simulink model "afe_inv_ttype_psm"  (R2026a)
settings: Solver=ode23tb  StopTime=simlength  FixedStep=tc  MaxStep=glb_time.tc
values from neighbouring files (symbols this model uses):
  afe_ctrl = ctrl_afe_setup(glb_time.ts_afe, grid_emu.omega_grid_nom)    [init_model.m]
  afe_pwm_phase_shift_mod1 = 0    [init_model.m]
  DThs_init = 0    [init_model.m]
  filters = setup_global_filters(glb_time.ts_afe, glb_time.ts_inv, glb_time.ts_dab, glb_time.tc)    [init_model.m]
  frt_data = frt_settings(test_index, test_subindex, asymmetric_error_type,      enable_frt_1, enable_frt_2, start_time_LVRT, deepPOSxi, deepPOSeta, deepNEGxi, deepNEGeta)    [init_model.m]
  glb_time = timing_setup(fpwm_afe, trgo_afe, fpwm_inv, trgo_inv, fpwm_single_phase_inv, trgo_single_phase_inv, fpwm_dab, trgo_dab,      fpwm_psfbc, trgo_psfbc, fpwm_isop_rail, trgo_isop_rail, fpwm_cllc, trgo_cllc, t_measure, tc_factor, tc_decimation, delay_pwm, dead_time_afe,      dead_time_inv, dead_time_single_phase_inv, dead_time_dab, dead_time_psfbc, dead_time_isop_rail, dead_time_cllc)    [init_model.m]
  grid_emu = grid_three_phase_emulator('Dyn11', delta_star, grid_nominal_power, application_voltage, us1, us2, fgrid,                  eq_grid_inductance, eq_grid_resistance, eta, ucc, i1m, p_iron, n1, n2, core_area, core_length, mur,                  up_xi_pu_ref, up_eta_pu_ref, un_xi_pu_ref, un_eta_pu_ref)    [init_model.m]
  i_react_pos_ref_2 = -ixi_ref_mod1*tan(acos(0.95))    [init_model.m]
  i_react_pos_ref_3 = ixi_ref_mod1*tan(acos(0.95))    [init_model.m]
  ixi_ref_mod1 = -0.85    [init_model.m]
  ki_align = 18    [init_model.m]
  kp_align = 0.25    [init_model.m]
  lim_down_align = -0.05    [init_model.m]
  lim_up_align = 0.05    [init_model.m]
  mavarage_filter_frequency_base_order = 2    [init_model.m]
  omega_m_sim = psm.omega_m_bez    [init_model.m]
  psm = psm_calculus()    [init_model.m]
  psm_ctrl = ctrl_pmsm_setup(glb_time.ts_inv, psm.omega_bez, u_psm_scale, psm.Jm_norm)    [init_model.m]
  simlength = 1.75    [init_model.m]
  Tambient = 40    [init_model.m]
  time_aux_power_supply_fault = 1e3    (= 1000)    [init_model.m]
  time_gain_afe_module_1 = 1.0002    [init_model.m]
  time_gain_inv_module_2 = 1.001    [init_model.m]
  time_i_react_pos_ref_1 = start_time_LVRT + error_length + 0.335    [init_model.m]
  time_i_react_pos_ref_2 = time_i_react_pos_ref_1 + 0.5    (= 0.5)    [init_model.m]
  time_start_motor_control = 0.25    [init_model.m]
  torque_overload_factor = 1    [init_model.m]
  u_cm_comp_mod1 = 0    [init_model.m]
  u_psm_scale_ekf = sqrt(3)/2 * 2/3 * hwdata.inv.udc_nom/psm.ubez    [init_model.m]
undefined symbols (not defined in the file or in its folder): hwdata, magnitude, omega_m_bez, rpm_base, torque_base
libraries: fl_lib x74, nesl_utility x43, moving_average_filter x10, moving_average_filter_cc x8, discrete_time_low_pass_filter x4, sl_discontinuities x3, single_phase_transformer_lib x3, linear_double_integrator_observer_ccaller x2, threephase_inductor_lib x2, dclink_for_three_levels x2, three_phase_three_level_ttype_inverter_ideal_switch_based_model x2, cstblocks_lti x2
(part 1 of 9)
settings Model: SimulationMode=accelerator  Creator=dbagn  LastModifiedBy=dbagn
settings SolverCC: NumberNewtonIterations=3.0  ZeroCrossControl=DisableAll  SolverResetMethod=Robust
settings SFSimCC: CustomCodeUndefinedFunction=ThrowError  DefaultCustomCodeDeterministicFunctions=All
settings SFSimCC: SimCustomHeaderCode=|
  | #include "rpi.h"
  | #include "mavgflt.h"
  | #include "mavgflt_simulink.h"
  | #include "mavgflts.h"
  | #include "mavgflts_simulink.h"
  | #include "dsmavgflt.h"
  | #include "dsmavgflt_simulink.h"
  | #include "bemf_obsv.h"
  | #include "bemf_obsv_simulink.h"
  | #include "bemf_obsv_load_est.h"
  | #include "bemf_obsv_load_est_simulink.h"
  | #include "dqvector_pi.h"
  | #include "dqvector_pi_simulink.h"
  | #include "sv_pwm_simulink.h"
  | #include "sv_pwm.h"
  | #include "sv_pwm_cm_simulink.h"
  | #include "sv_pwm_cm.h"
  | #include "first_harmonic_tracker.h"
  | #include "first_harmonic_tracker_simulink.h"
  | #include "dqpll_thyr.h"
  | #include "dqpll_thyr_simulink.h"
  | #include "dqpll_grid.h"
  | #include "dqpll_grid_simulink.h"
  | #include "linear_double_integrator_observer_simulink.h"
  | #include "linear_double_integrator_observer.h"
settings SFSimCC: SimUserSources=|
  | "rpi.c"
  | "mavgflt_simulink.c"
  | "mavgflt.c"
  | "mavgflts_simulink.c"
  | "mavgflts.c"
  | "dsmavgflt_simulink.c"
  | "dsmavgflt.c"
  | "bemf_obsv_simulink.c"
  | "bemf_obsv.c"
  | "bemf_obsv_load_est_simulink.c"
  | "bemf_obsv_load_est.c"
  | "dqvector_pi.c"
  | "dqvector_pi_simulink.c"
  | "sv_pwm_simulink.c"
  | "sv_pwm.c"
  | "sv_pwm_cm_simulink.c"
  | "sv_pwm_cm.c"
  | "first_harmonic_tracker_simulink.c"
  | "first_harmonic_tracker.c"
  | "dqpll_thyr_simulink.c"
  | "dqpll_thyr.c"
  | "dqpll_grid_simulink.c"
  | "dqpll_grid.c"
  | "linear_double_integrator_observer_simulink.c"
  | "linear_double_integrator_observer.c"
settings SFSimCC: SimUserIncludeDirs=|
  | include
  | src
settings SimscapeCC: SimscapeNominalValues="[{\"value\":\"1\",\"unit\":\"A\"},{\"value\":\"1\",\"unit\":\"bar\"},{\"value\":\"1\",\"unit\":\"cm^2\"},{\"value\":\"1\",\"unit\":\"cm^3/s\"},{\"value\":\"1\",\"unit\":\"kJ/kg\"},{\"value\":\"1\",\"unit\":\"kW\"},{\"value\":\"1\",\"unit\":\"l\"},{\"value\":\"1\",\"unit\":\"N\"},{\"value\":\"1\",\"unit\":\"N*m\"},{\"value\":\"1\",\"unit\":\"V\"}]"  SimscapeLogType=none  SimscapeLogDataHistory=5000.0

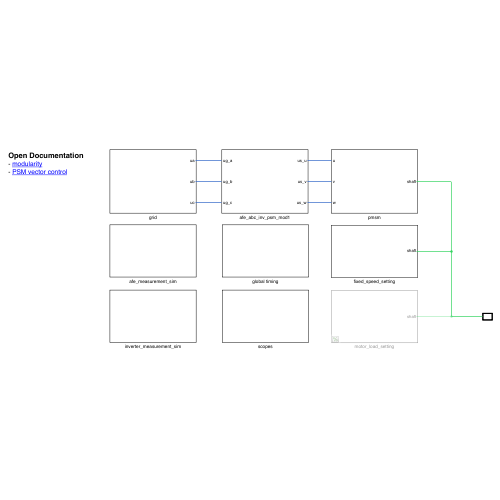
[thumbnail: Simulink's stored preview of the top-level diagram]
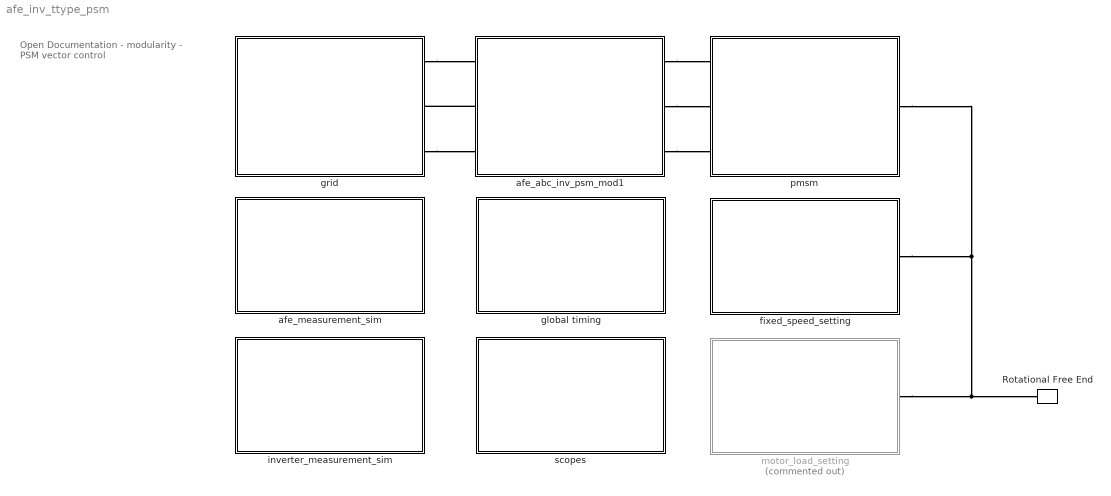
== system afe_inv_ttype_psm ==
  note: Open Documentation
      | - modularity
      | - PSM vector control
  Rotational Free End : fl_lib/Mechanical/Rotational Elements/Rotational Free End  w_specify=off  w_priority=None  w=0 rad/s  w_nominal_specify=off  w_nominal_value=1  w_nominal_unit=rad/s
  afe_abc_inv_psm_mod1 : Subsystem
  afe_measurement_sim : Subsystem
  fixed_speed_setting : Subsystem
  global timing : Subsystem
  grid : Subsystem
  inverter_measurement_sim : Subsystem
  motor_load_setting : Subsystem  Commented=on
  pmsm : Subsystem
  scopes : Subsystem
  connections:
  pmsm/RConn1 -- motor_load_setting/LConn1 -- Rotational Free End/LConn1 -- fixed_speed_setting/LConn1
  grid/RConn1 -- afe_abc_inv_psm_mod1/LConn1
  grid/RConn3 -- afe_abc_inv_psm_mod1/LConn3
  afe_abc_inv_psm_mod1/LConn2 -- grid/RConn2
  afe_abc_inv_psm_mod1/RConn2 -- pmsm/LConn2
  afe_abc_inv_psm_mod1/RConn1 -- pmsm/LConn1
  afe_abc_inv_psm_mod1/RConn3 -- pmsm/LConn3

== system afe_inv_ttype_psm/afe_abc_inv_psm_mod1 ==
  AFE_control : Subsystem
  LCL_filter : Subsystem
  afe : Subsystem
  brake : Subsystem
  inv_psm_mod1 : Subsystem
  ug_a : PMIOPort  Side=Left
  us_u : PMIOPort  Port=2  Side=Right
  ug_b : PMIOPort  Port=3  Side=Left
  us_v : PMIOPort  Port=4  Side=Right
  ug_c : PMIOPort  Port=5  Side=Left
  us_w : PMIOPort  Port=6  Side=Right
  wires:
  AFE_control/1(dabc_out) -> afe/1(dabc)
  connections:
  LCL_filter/LConn1 -- afe/LConn1
  LCL_filter/LConn2 -- afe/LConn2
  LCL_filter/LConn3 -- afe/LConn3
  LCL_filter/RConn1 -- ug_a/RConn1
  LCL_filter/RConn2 -- ug_b/RConn1
  LCL_filter/RConn3 -- ug_c/RConn1
  us_u/RConn1 -- inv_psm_mod1/RConn1
  us_v/RConn1 -- inv_psm_mod1/RConn2
  us_w/RConn1 -- inv_psm_mod1/RConn3
  inv_psm_mod1/LConn2 -- afe/RConn2
  afe/RConn1 -- brake/LConn1 -- inv_psm_mod1/LConn1
  afe/RConn3 -- brake/LConn2 -- inv_psm_mod1/LConn3

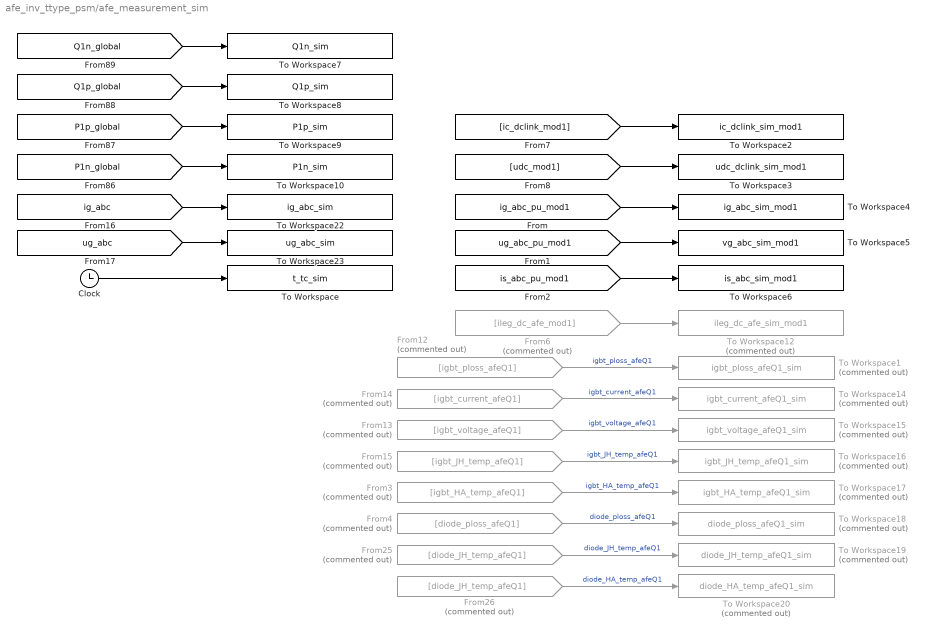
== system afe_inv_ttype_psm/afe_measurement_sim ==
  Clock : Clock
  From12 : From  Commented=on  GotoTag=igbt_ploss_afeQ1
  From13 : From  Commented=on  GotoTag=igbt_voltage_afeQ1
  From14 : From  Commented=on  GotoTag=igbt_current_afeQ1
  From15 : From  Commented=on  GotoTag=igbt_JH_temp_afeQ1
  From25 : From  Commented=on  GotoTag=diode_JH_temp_afeQ1
  From26 : From  Commented=on  GotoTag=diode_JH_temp_afeQ1
  From3 : From  Commented=on  GotoTag=igbt_HA_temp_afeQ1
  From4 : From  Commented=on  GotoTag=diode_ploss_afeQ1
  From6 : From  Commented=on  GotoTag=ileg_dc_afe_mod1
  To Workspace : ToWorkspace  VariableName=t_tc_sim  SampleTime=glb_time.tc
      settings: MaxDataPoints=glb_time.Nc
  To Workspace1 : ToWorkspace  Commented=on  VariableName=igbt_ploss_afeQ1_sim  SampleTime=glb_time.tc
      settings: MaxDataPoints=glb_time.Nc
  To Workspace10 : ToWorkspace  VariableName=P1n_sim  SampleTime=glb_time.ts_afe
      settings: MaxDataPoints=glb_time.Ns_afe
  To Workspace12 : ToWorkspace  Commented=on  VariableName=ileg_dc_afe_sim_mod1  SampleTime=glb_time.tc
      settings: MaxDataPoints=glb_time.Nc
  To Workspace14 : ToWorkspace  Commented=on  VariableName=igbt_current_afeQ1_sim  SampleTime=glb_time.tc
      settings: MaxDataPoints=glb_time.Nc
  To Workspace15 : ToWorkspace  Commented=on  VariableName=igbt_voltage_afeQ1_sim  SampleTime=glb_time.tc
      settings: MaxDataPoints=glb_time.Nc
  To Workspace16 : ToWorkspace  Commented=on  VariableName=igbt_JH_temp_afeQ1_sim  SampleTime=glb_time.tc
      settings: MaxDataPoints=glb_time.Nc
  To Workspace17 : ToWorkspace  Commented=on  VariableName=igbt_HA_temp_afeQ1_sim  SampleTime=glb_time.tc
      settings: MaxDataPoints=glb_time.Nc
  To Workspace18 : ToWorkspace  Commented=on  VariableName=diode_ploss_afeQ1_sim  SampleTime=glb_time.tc
      settings: MaxDataPoints=glb_time.Nc
  To Workspace19 : ToWorkspace  Commented=on  VariableName=diode_JH_temp_afeQ1_sim  SampleTime=glb_time.tc
      settings: MaxDataPoints=glb_time.Nc
  To Workspace2 : ToWorkspace  VariableName=ic_dclink_sim_mod1  SampleTime=glb_time.tc
      settings: MaxDataPoints=glb_time.Nc
  To Workspace20 : ToWorkspace  Commented=on  VariableName=diode_HA_temp_afeQ1_sim  SampleTime=glb_time.tc
      settings: MaxDataPoints=glb_time.Nc
  To Workspace22 : ToWorkspace  VariableName=ig_abc_sim  SampleTime=glb_time.tc
      settings: MaxDataPoints=glb_time.Nc
  To Workspace23 : ToWorkspace  VariableName=ug_abc_sim  SampleTime=glb_time.tc
      settings: MaxDataPoints=glb_time.Nc
  To Workspace3 : ToWorkspace  VariableName=udc_dclink_sim_mod1  SampleTime=glb_time.tc
      settings: MaxDataPoints=glb_time.Nc
  To Workspace4 : ToWorkspace  VariableName=ig_abc_sim_mod1  SampleTime=glb_time.tc
      settings: MaxDataPoints=glb_time.Nc
  To Workspace5 : ToWorkspace  VariableName=vg_abc_sim_mod1  SampleTime=glb_time.tc
      settings: MaxDataPoints=glb_time.Nc
  To Workspace6 : ToWorkspace  VariableName=is_abc_sim_mod1  SampleTime=glb_time.tc
      settings: MaxDataPoints=glb_time.Nc
  To Workspace7 : ToWorkspace  VariableName=Q1n_sim  SampleTime=glb_time.ts_afe
      settings: MaxDataPoints=glb_time.Ns_afe
  To Workspace8 : ToWorkspace  VariableName=Q1p_sim  SampleTime=glb_time.ts_afe
      settings: MaxDataPoints=glb_time.Ns_afe
  To Workspace9 : ToWorkspace  VariableName=P1p_sim  SampleTime=glb_time.ts_afe
      settings: MaxDataPoints=glb_time.Ns_afe
  wires:
  Clock/1 -> To Workspace/1
  [Q1n_global] -> To Workspace7/1
  [Q1p_global] -> To Workspace8/1
  [P1p_global] -> To Workspace9/1
  [P1n_global] -> To Workspace10/1
  [ug_abc] -> To Workspace23/1
  [ig_abc] -> To Workspace22/1
  [ug_abc_pu_mod1] -> To Workspace5/1
  [ig_abc_pu_mod1] -> To Workspace4/1
  From6/1 -> To Workspace12/1
  [udc_mod1] -> To Workspace3/1
  [ic_dclink_mod1] -> To Workspace2/1
  [is_abc_pu_mod1] -> To Workspace6/1
  From13/1 -> To Workspace15/1  "igbt_voltage_afeQ1"
  From3/1 -> To Workspace17/1  "igbt_HA_temp_afeQ1"
  From4/1 -> To Workspace18/1  "diode_ploss_afeQ1"
  From25/1 -> To Workspace19/1  "diode_JH_temp_afeQ1"
  From12/1 -> To Workspace1/1  "igbt_ploss_afeQ1"
  From26/1 -> To Workspace20/1  "diode_HA_temp_afeQ1"
  From14/1 -> To Workspace14/1  "igbt_current_afeQ1"
  From15/1 -> To Workspace16/1  "igbt_JH_temp_afeQ1"

== system afe_inv_ttype_psm/fixed_speed_setting ==
  Ideal Angular Velocity Source : fl_lib/Mechanical/Mechanical Sources/Ideal Angular Velocity Source
  Mechanical Rotational Reference : fl_lib/Mechanical/Rotational Elements/Mechanical Rotational Reference
  PS Step1 : fl_lib/Physical Signals/Sources/PS Step  step_time=0.025 s  initial_value=0 rpm  final_value=rpm_sim rpm
  PS Transfer Function : fl_lib/Physical Signals/Linear Operators/PS Transfer Function  transfer_function_type=foundation.enum.transfer_function_type.lag  T=0.1 s  T1=2 s  T2=1 s  reset_method=foundation.enum.IntegratorResetSpec.None  initial_condition_spec=foundation.enum.IntegratorICSpec.Internal  y0=0 rpm
  shaft : PMIOPort  Side=Left
  connections:
  Mechanical Rotational Reference/LConn1 -- Ideal Angular Velocity Source/RConn2
  PS Step1/RConn1 -- PS Transfer Function/LConn1
  PS Transfer Function/RConn1 -- Ideal Angular Velocity Source/RConn1
  Ideal Angular Velocity Source/LConn1 -- shaft/RConn1

== system afe_inv_ttype_psm/global timing ==
  Unit Delay : UnitDelay  SampleTime=glb_time.tc
  Unit Delay1 : UnitDelay  SampleTime=glb_time.tc
  time_afe1 : Subsystem  mask{k=time_gain_afe_module_1}
      mask prompts: k "Time Gain"
      mask Display:
      | disp('time-gen');
      | port_label('input', 1, 'crt');
      | port_label('output', 1, 'tout');
  time_afe3 : Subsystem  mask{k=1}
      mask prompts: k "Time Gain"
      mask Display:
      | disp('time-gen');
      | port_label('output', 1, 'tout');
  time_inv1 : Subsystem  mask{k=time_gain_inv_module_2}
      mask prompts: k "Time Gain"
      mask Display:
      | disp('time-gen');
      | port_label('input', 1, 'crt');
      | port_label('output', 1, 'tout');
  tag scope: time_afe_module_1=global, time_inv_module_1=global, time_master=global
  wires:
  time_afe1/1(Out1) -> [time_afe_module_1]
  time_inv1/1(Out1) -> [time_inv_module_1]
  time_afe3/1(Out1) -> [time_master]
  [local_time_corr_afe1] -> Unit Delay/1
  Unit Delay/1 -> time_afe1/1(correction_time)
  [local_time_corr_inv1] -> Unit Delay1/1
  Unit Delay1/1 -> time_inv1/1(correction_time)

== system afe_inv_ttype_psm/grid ==
  Bus Selector : BusSelector  OutputSignals=Q1p,Q1n,P1n,P1p,U1n,U1p,i_act_1n,i_react_1n,i_act_1p,i_react_1p
  To Workspace1 : ToWorkspace  VariableName=i_react_1n  SampleTime=glb_time.ts_afe
      settings: MaxDataPoints=glb_time.Ns_afe
  To Workspace2 : ToWorkspace  VariableName=i_react_1p  SampleTime=glb_time.ts_afe
      settings: MaxDataPoints=glb_time.Ns_afe
  To Workspace3 : ToWorkspace  VariableName=i_act_1n  SampleTime=glb_time.ts_afe
      settings: MaxDataPoints=glb_time.Ns_afe
  To Workspace4 : ToWorkspace  VariableName=i_act_1p  SampleTime=glb_time.ts_afe
      settings: MaxDataPoints=glb_time.Ns_afe
  To Workspace5 : ToWorkspace  VariableName=u1p  SampleTime=glb_time.ts_afe
      settings: MaxDataPoints=glb_time.Ns_afe
  To Workspace6 : ToWorkspace  VariableName=u1n  SampleTime=glb_time.ts_afe
      settings: MaxDataPoints=glb_time.Ns_afe
  grid_emulator : Subsystem
  power meter iec : power_meter_iec/power meter iec  period=pi/grid_emu.omega_grid_nom  ts=glb_time.ts_afe  enable_time=0.025
  threephase_vi_measures : Subsystem
  ua : PMIOPort  Side=Right
  ub : PMIOPort  Port=2  Side=Right
  uc : PMIOPort  Port=3  Side=Right
  tag scope: P1n_global=global, P1p_global=global, Q1n_global=global, Q1p_global=global
  wires:
  [gamma_grid_emulator] -> power meter iec/1
  [ug_abc] -> power meter iec/2
  [ig_abc] -> power meter iec/3
  power meter iec/1 -> Bus Selector/1
  Bus Selector/1 -> [Q1p_global]  "<Q1p>"
  Bus Selector/2 -> [Q1n_global]  "<Q1n>"
  Bus Selector/3 -> [P1n_global]  "<P1n>"
  Bus Selector/4 -> [P1p_global]  "<P1p>"
  Bus Selector/5 -> To Workspace6/1  "<U1n>"
  Bus Selector/6 -> To Workspace5/1  "<U1p>"
  Bus Selector/7 -> To Workspace3/1  "<i_act_1n>"
  Bus Selector/8 -> To Workspace1/1  "<i_react_1n>"
  Bus Selector/9 -> To Workspace4/1  "<i_act_1p>"
  Bus Selector/10 -> To Workspace2/1  "<i_react_1p>"
  [omega_grid_emulator] -> power meter iec/4
  connections:
  threephase_vi_measures/LConn3 -- grid_emulator/RConn3
  threephase_vi_measures/LConn1 -- grid_emulator/RConn1
  threephase_vi_measures/RConn2 -- ub/RConn1
  threephase_vi_measures/LConn2 -- grid_emulator/RConn2
  threephase_vi_measures/RConn1 -- ua/RConn1
  threephase_vi_measures/RConn3 -- uc/RConn1

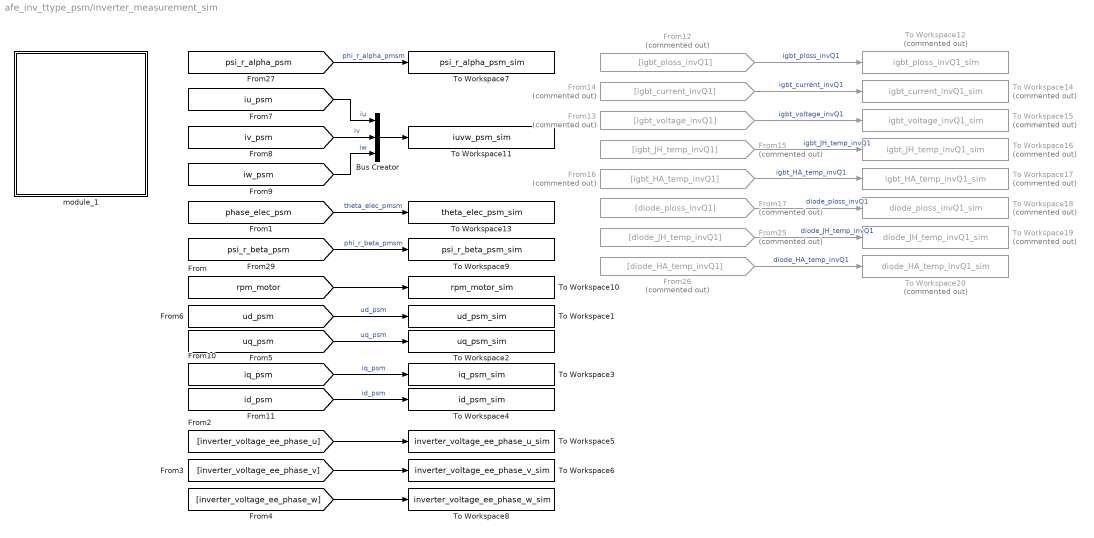
== system afe_inv_ttype_psm/inverter_measurement_sim ==
  Bus Creator : BusCreator  Inputs=3
  From12 : From  Commented=on  GotoTag=igbt_ploss_invQ1
  From13 : From  Commented=on  GotoTag=igbt_voltage_invQ1
  From14 : From  Commented=on  GotoTag=igbt_current_invQ1
  From15 : From  Commented=on  GotoTag=igbt_JH_temp_invQ1
  From16 : From  Commented=on  GotoTag=igbt_HA_temp_invQ1
  From17 : From  Commented=on  GotoTag=diode_ploss_invQ1
  From25 : From  Commented=on  GotoTag=diode_JH_temp_invQ1
  From26 : From  Commented=on  GotoTag=diode_HA_temp_invQ1
  To Workspace1 : ToWorkspace  VariableName=ud_psm_sim  SampleTime=glb_time.tc
      settings: MaxDataPoints=glb_time.Nc
  To Workspace10 : ToWorkspace  VariableName=rpm_motor_sim  SampleTime=glb_time.tc
      settings: MaxDataPoints=glb_time.Nc
  To Workspace11 : ToWorkspace  VariableName=iuvw_psm_sim  SampleTime=glb_time.tc
      settings: MaxDataPoints=glb_time.Nc
  To Workspace12 : ToWorkspace  Commented=on  VariableName=igbt_ploss_invQ1_sim  SampleTime=glb_time.tc
      settings: MaxDataPoints=glb_time.Nc
  To Workspace13 : ToWorkspace  VariableName=theta_elec_psm_sim  SampleTime=glb_time.tc
      settings: MaxDataPoints=glb_time.Nc
  To Workspace14 : ToWorkspace  Commented=on  VariableName=igbt_current_invQ1_sim  SampleTime=glb_time.tc
      settings: MaxDataPoints=glb_time.Nc
  To Workspace15 : ToWorkspace  Commented=on  VariableName=igbt_voltage_invQ1_sim  SampleTime=glb_time.tc
      settings: MaxDataPoints=glb_time.Nc
  To Workspace16 : ToWorkspace  Commented=on  VariableName=igbt_JH_temp_invQ1_sim  SampleTime=glb_time.tc
      settings: MaxDataPoints=glb_time.Nc
  To Workspace17 : ToWorkspace  Commented=on  VariableName=igbt_HA_temp_invQ1_sim  SampleTime=glb_time.tc
      settings: MaxDataPoints=glb_time.Nc
  To Workspace18 : ToWorkspace  Commented=on  VariableName=diode_ploss_invQ1_sim  SampleTime=glb_time.tc
      settings: MaxDataPoints=glb_time.Nc
  To Workspace19 : ToWorkspace  Commented=on  VariableName=diode_JH_temp_invQ1_sim  SampleTime=glb_time.tc
      settings: MaxDataPoints=glb_time.Nc
  To Workspace2 : ToWorkspace  VariableName=uq_psm_sim  SampleTime=glb_time.tc
      settings: MaxDataPoints=glb_time.Nc
  To Workspace20 : ToWorkspace  Commented=on  VariableName=diode_HA_temp_invQ1_sim  SampleTime=glb_time.tc
      settings: MaxDataPoints=glb_time.Nc
  To Workspace3 : ToWorkspace  VariableName=iq_psm_sim  SampleTime=glb_time.tc
      settings: MaxDataPoints=glb_time.Nc
  To Workspace4 : ToWorkspace  VariableName=id_psm_sim  SampleTime=glb_time.tc
      settings: MaxDataPoints=glb_time.Nc
  To Workspace5 : ToWorkspace  VariableName=inverter_voltage_ee_phase_u_sim  SampleTime=glb_time.tc
      settings: MaxDataPoints=glb_time.Nc
  To Workspace6 : ToWorkspace  VariableName=inverter_voltage_ee_phase_v_sim  SampleTime=glb_time.tc
      settings: MaxDataPoints=glb_time.Nc
  To Workspace7 : ToWorkspace  VariableName=psi_r_alpha_psm_sim  SampleTime=glb_time.tc
      settings: MaxDataPoints=glb_time.Nc
  To Workspace8 : ToWorkspace  VariableName=inverter_voltage_ee_phase_w_sim  SampleTime=glb_time.tc
      settings: MaxDataPoints=glb_time.Nc
  To Workspace9 : ToWorkspace  VariableName=psi_r_beta_psm_sim  SampleTime=glb_time.tc
      settings: MaxDataPoints=glb_time.Nc
  module_1 : Subsystem
  wires:
  [psi_r_alpha_psm] -> To Workspace7/1  "phi_r_alpha_pmsm"
  [psi_r_beta_psm] -> To Workspace9/1  "phi_r_beta_pmsm"
  [rpm_motor] -> To Workspace10/1
  [iv_psm] -> Bus Creator/2  "iv"
  [iw_psm] -> Bus Creator/3  "iw"
  [iu_psm] -> Bus Creator/1  "iu"
  Bus Creator/1 -> To Workspace11/1
  [phase_elec_psm] -> To Workspace13/1  "theta_elec_pmsm"
  [ud_psm] -> To Workspace1/1  "ud_psm"
  [uq_psm] -> To Workspace2/1  "uq_psm"
  [iq_psm] -> To Workspace3/1  "iq_psm"
  [id_psm] -> To Workspace4/1  "id_psm"
  [inverter_voltage_ee_phase_u] -> To Workspace5/1
  [inverter_voltage_ee_phase_v] -> To Workspace6/1
  [inverter_voltage_ee_phase_w] -> To Workspace8/1
  From26/1 -> To Workspace20/1  "diode_HA_temp_invQ1"
  From14/1 -> To Workspace14/1  "igbt_current_invQ1"
  From17/1 -> To Workspace18/1  "diode_ploss_invQ1"
  From25/1 -> To Workspace19/1  "diode_JH_temp_invQ1"
  From16/1 -> To Workspace17/1  "igbt_HA_temp_invQ1"
  From12/1 -> To Workspace12/1  "igbt_ploss_invQ1"
  From13/1 -> To Workspace15/1  "igbt_voltage_invQ1"
  From15/1 -> To Workspace16/1  "igbt_JH_temp_invQ1"

== system afe_inv_ttype_psm/motor_load_setting ==
  Ideal Torque Source : fl_lib/Mechanical/Mechanical Sources/Ideal Torque Source
  Inertia : fl_lib/Mechanical/Rotational Elements/Inertia  inertia=external_load_inertia kg*m^2  num_ports=foundation.enum.numPorts2.one  w_specify=off  w_priority=High  w=0 rad/s  w_nominal_specify=off  w_nominal_value=1  w_nominal_unit=rad/s  t_specify=off  t_priority=None  t=0 N*m  t_nominal_specify=off  t_nominal_value=1  t_nominal_unit=N*m
  Mechanical Rotational Reference : fl_lib/Mechanical/Rotational Elements/Mechanical Rotational Reference
  PS Step : fl_lib/Physical Signals/Sources/PS Step  step_time=load_step_time s  initial_value=1 N*m  final_value=1 N*m
  PS Transfer Function : fl_lib/Physical Signals/Linear Operators/PS Transfer Function  transfer_function_type=foundation.enum.transfer_function_type.lag  T=1 s  T1=2 s  T2=1 s  reset_method=foundation.enum.IntegratorResetSpec.None  initial_condition_spec=foundation.enum.IntegratorICSpec.Internal  y0=0 N*m
  flexible_shaft : simple_flexible_shaft/flexible_shaft  b1=1  b2=1  J1=1  J2=1  b_displacement=1  k_displacement=1e5
  shaft : PMIOPort  Side=Left
  connections:
  Ideal Torque Source/LConn1 -- flexible_shaft/RConn1 -- Inertia/LConn1
  Ideal Torque Source/RConn2 -- Mechanical Rotational Reference/LConn1
  PS Transfer Function/RConn1 -- Ideal Torque Source/RConn1
  PS Step/RConn1 -- PS Transfer Function/LConn1
  flexible_shaft/LConn1 -- shaft/RConn1

== system afe_inv_ttype_psm/pmsm ==
  Bus Selector1 : BusSelector  OutputSignals=omega_mech (rpm)
  Constant : Constant  Value=psm.psi_m
  Simulink-PS Converter3 : nesl_utility/Simulink-PS Converter  PhysicalDomain=network_engine_domain  SubClassName=ps_input  LeftPortType=input  RightPortType=output  PseudoPeriodic=off  Frequencies=[]  NoiseDistribution=none  NoiseParameters=[]  Unit=V*s  AffineConversion=on  FilteringAndDerivatives=provide  SimscapeFilterOrder=1  InputFilterTimeConstant=0.001  UdotUserProvided=0
  synchronous_motor : Subsystem
  u : PMIOPort  Side=Left
  v : PMIOPort  Port=2  Side=Left
  w : PMIOPort  Port=3  Side=Left
  shaft : PMIOPort  Port=4  Side=Right
  tag scope: rpm_motor=global
  wires:
  synchronous_motor/1(motor_data) -> Bus Selector1/1
  Bus Selector1/1 -> [rpm_motor]  "<omega_mech (rpm)>"
  Constant/1 -> Simulink-PS Converter3/1
  connections:
  synchronous_motor/LConn1 -- u/RConn1
  Simulink-PS Converter3/RConn1 -- synchronous_motor/LConn4
  synchronous_motor/LConn3 -- w/RConn1
  synchronous_motor/LConn2 -- v/RConn1
  shaft/RConn1 -- synchronous_motor/RConn1

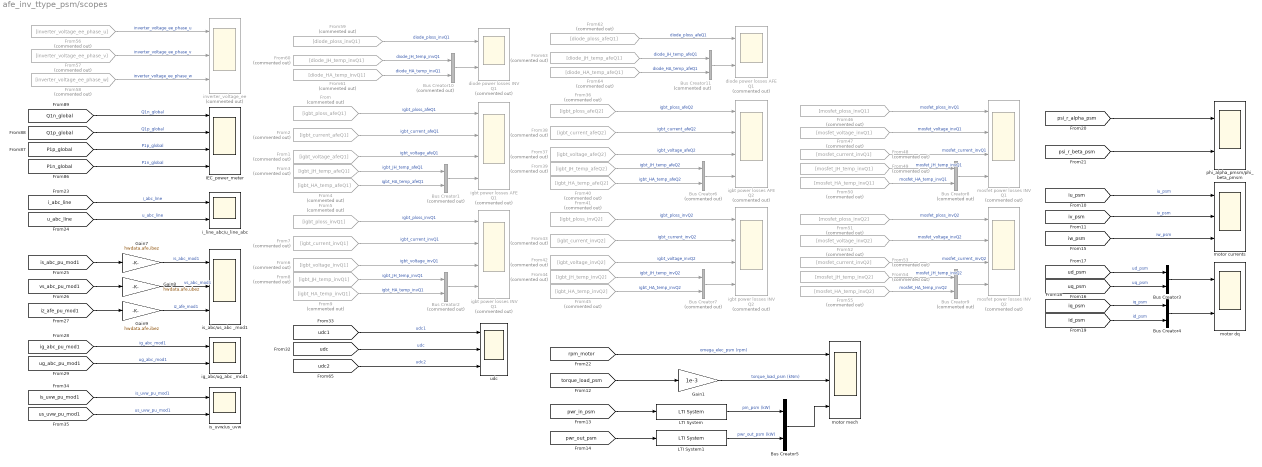
== system afe_inv_ttype_psm/scopes ==
  Bus Creator{1..2,6..11} (8 alike) : BusCreator  Commented=on  Inputs=2
  Bus Creator3 : BusCreator  Inputs=2
  Bus Creator4 : BusCreator  Inputs=2
  Bus Creator5 : BusCreator  Inputs=2
  From : From  Commented=on  GotoTag=igbt_ploss_afeQ1
  From1 : From  Commented=on  GotoTag=igbt_voltage_afeQ1
  From2 : From  Commented=on  GotoTag=igbt_current_afeQ1
  From3 : From  Commented=on  GotoTag=igbt_JH_temp_afeQ1
  From36 : From  Commented=on  GotoTag=igbt_ploss_afeQ2
  From37 : From  Commented=on  GotoTag=igbt_voltage_afeQ2
  From38 : From  Commented=on  GotoTag=igbt_current_afeQ2
  From39 : From  Commented=on  GotoTag=igbt_JH_temp_afeQ2
  From4 : From  Commented=on  GotoTag=igbt_HA_temp_afeQ1
  From40 : From  Commented=on  GotoTag=igbt_HA_temp_afeQ2
  From41 : From  Commented=on  GotoTag=igbt_ploss_invQ2
  From42 : From  Commented=on  GotoTag=igbt_voltage_invQ2
  From43 : From  Commented=on  GotoTag=igbt_current_invQ2
  From44 : From  Commented=on  GotoTag=igbt_JH_temp_invQ2
  From45 : From  Commented=on  GotoTag=igbt_HA_temp_invQ2
  From46 : From  Commented=on  GotoTag=mosfet_ploss_invQ1
  From47 : From  Commented=on  GotoTag=mosfet_voltage_invQ1
  From48 : From  Commented=on  GotoTag=mosfet_current_invQ1
  From49 : From  Commented=on  GotoTag=mosfet_JH_temp_invQ1
  From5 : From  Commented=on  GotoTag=igbt_ploss_invQ1
  From50 : From  Commented=on  GotoTag=mosfet_HA_temp_invQ1
  From51 : From  Commented=on  GotoTag=mosfet_ploss_invQ2
  From52 : From  Commented=on  GotoTag=mosfet_voltage_invQ2
  From53 : From  Commented=on  GotoTag=mosfet_current_invQ2
  From54 : From  Commented=on  GotoTag=mosfet_JH_temp_invQ2
  From55 : From  Commented=on  GotoTag=mosfet_HA_temp_invQ2
  From56 : From  Commented=on  GotoTag=inverter_voltage_ee_phase_u
  From57 : From  Commented=on  GotoTag=inverter_voltage_ee_phase_v
  From58 : From  Commented=on  GotoTag=inverter_voltage_ee_phase_w
  From59 : From  Commented=on  GotoTag=diode_ploss_invQ1
  From6 : From  Commented=on  GotoTag=igbt_voltage_invQ1
  From60 : From  Commented=on  GotoTag=diode_JH_temp_invQ1
  From61 : From  Commented=on  GotoTag=diode_HA_temp_invQ1
  From62 : From  Commented=on  GotoTag=diode_ploss_afeQ1
  From63 : From  Commented=on  GotoTag=diode_JH_temp_afeQ1
  From64 : From  Commented=on  GotoTag=diode_HA_temp_afeQ1
  From7 : From  Commented=on  GotoTag=igbt_current_invQ1
  From8 : From  Commented=on  GotoTag=igbt_JH_temp_invQ1
  From9 : From  Commented=on  GotoTag=igbt_HA_temp_invQ1
  Gain1 : Gain  Gain=1e-3
  Gain7 : Gain  Gain=hwdata.afe.ibez
  Gain8 : Gain  Gain=hwdata.afe.ubez
  Gain9 : Gain  Gain=hwdata.afe.ibez
  IEC_power_meter : Scope  NumInputPorts=4
      settings: ActiveDisplayYMinimum=-45629.81930074111  ActiveDisplayYMaximum=397375.85061644186  DataLoggingVariableName=ScopeData14
  LTI System : cstblocks_lti/LTI System  sys=filters.inv.SOF_50Hz.ss_c  IC=[]  PadeOrder=0
  LTI System1 : cstblocks_lti/LTI System  sys=filters.inv.SOF_50Hz.ss_c  IC=[]  PadeOrder=0
  diode power losses AFE Q1 : Scope  Commented=on  NumInputPorts=2
      settings: SampleTime=glb_time.tc  ActiveDisplayYMinimum=-0.87039317174009745  ActiveDisplayYMaximum=7.8312553964690395  DataLoggingVariableName=ScopeData32
  diode power losses INV Q1 : Scope  Commented=on  NumInputPorts=2
      settings: SampleTime=glb_time.tc  ActiveDisplayYMinimum=-1  ActiveDisplayYMaximum=1  DataLoggingVariableName=ScopeData31
  i_line_abc/u_line_abc : Scope  NumInputPorts=2
      settings: SampleTime=glb_time.tc  ActiveDisplayYMinimum=-1843.0536022673643  ActiveDisplayYMaximum=1951.2827711955147  DataLoggingVariableName=ScopeData20
  ig_abc/ug_abc _mod1 : Scope  NumInputPorts=2
      settings: SampleTime=glb_time.tc  ActiveDisplayYMinimum=-2.2818604167933909  ActiveDisplayYMaximum=2.3578077253605345  DataLoggingVariableName=ScopeData22
  igbt power losses AFE Q1 : Scope  Commented=on  NumInputPorts=4
      settings: SampleTime=glb_time.tc  ActiveDisplayYMinimum=-49.42236160670042  ActiveDisplayYMaximum=444.75917558996025  DataLoggingVariableName=ScopeData15
  igbt power losses AFE Q2 : Scope  Commented=on  NumInputPorts=4
      settings: SampleTime=glb_time.tc  ActiveDisplayYMinimum=-81.375120798865652  ActiveDisplayYMaximum=732.47476633188421  DataLoggingVariableName=ScopeData26
  igbt power losses INV Q1 : Scope  Commented=on  NumInputPorts=4
      settings: SampleTime=glb_time.tc  ActiveDisplayYMinimum=427.7171442031123  ActiveDisplayYMaximum=1026.5989043156007  DataLoggingVariableName=ScopeData16
  igbt power losses INV Q2 : Scope  Commented=on  NumInputPorts=4
      settings: SampleTime=glb_time.tc  ActiveDisplayYMinimum=-115137.16014702634  ActiveDisplayYMaximum=1.0362344192177997E+6  DataLoggingVariableName=ScopeData27
  inverter_voltage_ee : Scope  Commented=on  NumInputPorts=3
      settings: SampleTime=tc  ActiveDisplayYMinimum=-207.5782073641667  ActiveDisplayYMaximum=1301.7632755987056  DataLoggingVariableName=ScopeData30
  is_abc/us_abc _mod1 : Scope  NumInputPorts=3
      settings: SampleTime=glb_time.tc  ActiveDisplayYMinimum=-656.64544191213372  ActiveDisplayYMaximum=546.43356350725981  DataLoggingVariableName=ScopeData21
  is_uvw/us_uvw : Scope  NumInputPorts=2
      settings: SampleTime=glb_time.tc  ActiveDisplayYMinimum=-0.26533507295709952  ActiveDisplayYMaximum=0.2861938805031341  DataLoggingVariableName=ScopeData25
  mosfet power losses INV Q1 : Scope  Commented=on  NumInputPorts=4
      settings: SampleTime=glb_time.tc  ActiveDisplayYMinimum=-52.647210306071649  ActiveDisplayYMaximum=473.81757031333393  DataLoggingVariableName=ScopeData28
  mosfet power losses INV Q2 : Scope  Commented=on  NumInputPorts=4
      settings: SampleTime=glb_time.tc  ActiveDisplayYMinimum=-60.051099059926763  ActiveDisplayYMaximum=540.45256909803  DataLoggingVariableName=ScopeData29
  motor currents : Scope  NumInputPorts=3
      settings: SampleTime=glb_time.tc  ActiveDisplayYMinimum=-572.6153664757129  ActiveDisplayYMaximum=573.538162291844  DataLoggingVariableName=ScopeData17
  motor dq : Scope  NumInputPorts=2
      settings: SampleTime=glb_time.tc  ActiveDisplayYMinimum=-850.02239826316088  ActiveDisplayYMaximum=207.16586596148719  DataLoggingVariableName=ScopeData18
  motor mech : Scope  NumInputPorts=3
      settings: SampleTime=glb_time.tc  ActiveDisplayYMinimum=-2.2249893529432536  ActiveDisplayYMaximum=20.024904176489287  DataLoggingVariableName=ScopeData11
  phi_alpha_pmsm/phi_beta_pmsm : Scope  NumInputPorts=2
      settings: SampleTime=glb_time.tc  ActiveDisplayYMinimum=-4.8008048511588592  ActiveDisplayYMaximum=4.8008564448893649  DataLoggingVariableName=ScopeData19
  udc : Scope  NumInputPorts=3
      settings: SampleTime=glb_time.tc  ActiveDisplayYMinimum=-178.76888876516341  ActiveDisplayYMaximum=1609.2261461414053  DataLoggingVariableName=ScopeData23
  wires:
  [Q1p_global] -> IEC_power_meter/2  "Q1p_global"
  [P1n_global] -> IEC_power_meter/4  "P1n_global"
  [Q1n_global] -> IEC_power_meter/1  "Q1n_global"
  [P1p_global] -> IEC_power_meter/3  "P1p_global"
  From1/1 -> igbt power losses AFE Q1/3  "igbt_voltage_afeQ1"
  Bus Creator1/1 -> igbt power losses AFE Q1/4
  From/1 -> igbt power losses AFE Q1/1  "igbt_ploss_afeQ1"
  From4/1 -> Bus Creator1/2  "igbt_HA_temp_afeQ1"
  From3/1 -> Bus Creator1/1  "igbt_JH_temp_afeQ1"
  From2/1 -> igbt power losses AFE Q1/2  "igbt_current_afeQ1"
  From5/1 -> igbt power losses INV Q1/1  "igbt_ploss_invQ1"
  From7/1 -> igbt power losses INV Q1/2  "igbt_current_invQ1"
  From8/1 -> Bus Creator2/1  "igbt_JH_temp_invQ1"
  From9/1 -> Bus Creator2/2  "igbt_HA_temp_invQ1"
  Bus Creator2/1 -> igbt power losses INV Q1/4
  From6/1 -> igbt power losses INV Q1/3  "igbt_voltage_invQ1"
  [torque_load_psm] -> Gain1/1
  [pwr_out_psm] -> LTI System1/1
  Bus Creator4/1 -> motor dq/2
  LTI System/1 -> Bus Creator5/1  "pin_psm (kW)"
  LTI System1/1 -> Bus Creator5/2  "pwr_out_psm (kW)"
  [iw_psm] -> motor currents/3  "iw_psm"
  Gain1/1 -> motor mech/2  "torque_load_psm (kNm)"
  [id_psm] -> Bus Creator4/2  "id_psm"
  [psi_r_alpha_psm] -> phi_alpha_pmsm/phi_beta_pmsm/1
  [iv_psm] -> motor currents/2  "iv_psm"
  Bus Creator3/1 -> motor dq/1
  [uq_psm] -> Bus Creator3/2  "uq_psm"
  [iu_psm] -> motor currents/1  "iu_psm"
  Bus Creator5/1 -> motor mech/3
  [ud_psm] -> Bus Creator3/1  "ud_psm"
  [iq_psm] -> Bus Creator4/1  "iq_psm"
  [rpm_motor] -> motor mech/1  "omega_elec_psm (rpm)"
  [pwr_in_psm] -> LTI System/1
  [psi_r_beta_psm] -> phi_alpha_pmsm/phi_beta_pmsm/2
  [u_abc_line] -> i_line_abc/u_line_abc/2  "u_abc_line"
  [i_abc_line] -> i_line_abc/u_line_abc/1  "i_abc_line"
  Gain7/1 -> is_abc/us_abc _mod1/1  "is_abc_mod1"
  [is_abc_pu_mod1] -> Gain7/1
  [vs_abc_pu_mod1] -> Gain8/1
  [iz_afe_pu_mod1] -> Gain9/1
  Gain8/1 -> is_abc/us_abc _mod1/2  "vs_abc_mod1"
  Gain9/1 -> is_abc/us_abc _mod1/3  "iz_afe_mod1"
  [ig_abc_pu_mod1] -> ig_abc/ug_abc _mod1/1  "ig_abc_mod1"
  [ug_abc_pu_mod1] -> ig_abc/ug_abc _mod1/2  "ug_abc_mod1"
  [udc1] -> udc/1  "udc1"
  [udc] -> udc/2  "udc"
  [is_uvw_pu_mod1] -> is_uvw/us_uvw/1  "is_uvw_pu_mod1"
  [us_uvw_pu_mod1] -> is_uvw/us_uvw/2  "us_uvw_pu_mod1"
  From42/1 -> igbt power losses INV Q2/3  "igbt_voltage_invQ2"
  Bus Creator7/1 -> igbt power losses INV Q2/4
  From45/1 -> Bus Creator7/2  "igbt_HA_temp_invQ2"
  From44/1 -> Bus Creator7/1  "igbt_JH_temp_invQ2"
  From43/1 -> igbt power losses INV Q2/2  "igbt_current_invQ2"
  From41/1 -> igbt power losses INV Q2/1  "igbt_ploss_invQ2"
  From38/1 -> igbt power losses AFE Q2/2  "igbt_current_afeQ2"
  From39/1 -> Bus Creator6/1  "igbt_JH_temp_afeQ2"
  From40/1 -> Bus Creator6/2  "igbt_HA_temp_afeQ2"
  From36/1 -> igbt power losses AFE Q2/1  "igbt_ploss_afeQ2"
  Bus Creator6/1 -> igbt power losses AFE Q2/4
  From37/1 -> igbt power losses AFE Q2/3  "igbt_voltage_afeQ2"
  Bus Creator8/1 -> mosfet power losses INV Q1/4
  Bus Creator9/1 -> mosfet power losses INV Q2/4
  From46/1 -> mosfet power losses INV Q1/1  "mosfet_ploss_invQ1"
  From47/1 -> mosfet power losses INV Q1/2  "mosfet_voltage_invQ1"
  From51/1 -> mosfet power losses INV Q2/1  "mosfet_ploss_invQ2"
  From52/1 -> mosfet power losses INV Q2/2  "mosfet_voltage_invQ2"
  From53/1 -> mosfet power losses INV Q2/3  "mosfet_current_invQ2"
  From54/1 -> Bus Creator9/1  "mosfet_JH_temp_invQ2"
  From55/1 -> Bus Creator9/2  "mosfet_HA_temp_invQ2"
  From50/1 -> Bus Creator8/2  "mosfet_HA_temp_invQ1"
  From49/1 -> Bus Creator8/1  "mosfet_JH_temp_invQ1"
  From48/1 -> mosfet power losses INV Q1/3  "mosfet_current_invQ1"
  From56/1 -> inverter_voltage_ee/1  "inverter_voltage_ee_phase_u"
  From58/1 -> inverter_voltage_ee/3  "inverter_voltage_ee_phase_w"
  From57/1 -> inverter_voltage_ee/2  "inverter_voltage_ee_phase_v"
  From61/1 -> Bus Creator10/2  "diode_HA_temp_invQ1"
  From60/1 -> Bus Creator10/1  "diode_JH_temp_invQ1"
  Bus Creator10/1 -> diode power losses INV Q1/2
  From59/1 -> diode power losses INV Q1/1  "diode_ploss_invQ1"
  From62/1 -> diode power losses AFE Q1/1  "diode_ploss_afeQ1"
  Bus Creator11/1 -> diode power losses AFE Q1/2
  From63/1 -> Bus Creator11/1  "diode_JH_temp_afeQ1"
  From64/1 -> Bus Creator11/2  "diode_HA_temp_afeQ1"
  [udc2] -> udc/3  "udc2"

== system afe_inv_ttype_psm/afe_abc_inv_psm_mod1/AFE_control ==
  To Workspace : ToWorkspace  VariableName=afe_ctrl_data_output_mod1  SampleTime=glb_time.ts_afe
      settings: MaxDataPoints=glb_time.Ns_afe
  afe_control : Subsystem
  dabc_out : Outport
  tag scope: local_time_corr_afe1=global
  wires:
  [TRGO_afe_module_1] -> afe_control/Trigger
  [ug_abc_pu_mod1] -> afe_control/1(ug_abc_pu)
  [is_abc_pu_mod1] -> afe_control/4(is_abc_pu)
  [vdc_pu] -> afe_control/2(udc_pu)
  afe_control/1(duvw) -> dabc_out/1
  [ig_abc_pu_mod1] -> afe_control/3(ig_abc_pu)
  [time_afe_module_1] -> afe_control/5(local_time)
  [time_master] -> afe_control/6(master_time)
  afe_control/2(AFE1_local_time_corr) -> [local_time_corr_afe1]
  [gamma_grid_emulator] -> afe_control/7(grid_phase)
  afe_control/3(m_data) -> To Workspace/1

== system afe_inv_ttype_psm/afe_abc_inv_psm_mod1/LCL_filter ==
  CFu1 : fl_lib/Electrical/Electrical Elements/Capacitor  c=hwdata.afe.CFu F  r=hwdata.afe.RCFu Ohm  g=0 1/Ohm  i_specify=off  i_priority=None  i=0 A  i_nominal_specify=off  i_nominal_value=1  i_nominal_unit=A  v_specify=off  v_priority=None  v=0 V  v_nominal_specify=off  v_nominal_value=1  v_nominal_unit=V  vc_specify=off  vc_priority=High  vc=0 V  vc_nominal_specify=off  vc_nominal_value=1  vc_nominal_unit=V
  CFu2 : fl_lib/Electrical/Electrical Elements/Capacitor  c=hwdata.afe.CFu F  r=hwdata.afe.RCFu Ohm  g=0 1/Ohm  i_specify=off  i_priority=None  i=0 A  i_nominal_specify=off  i_nominal_value=1  i_nominal_unit=A  v_specify=off  v_priority=None  v=0 V  v_nominal_specify=off  v_nominal_value=1  v_nominal_unit=V  vc_specify=off  vc_priority=High  vc=0 V  vc_nominal_specify=off  vc_nominal_value=1  vc_nominal_unit=V
  CFu3 : fl_lib/Electrical/Electrical Elements/Capacitor  c=hwdata.afe.CFu F  r=hwdata.afe.RCFu Ohm  g=0 1/Ohm  i_specify=off  i_priority=None  i=0 A  i_nominal_specify=off  i_nominal_value=1  i_nominal_unit=A  v_specify=off  v_priority=None  v=0 V  v_nominal_specify=off  v_nominal_value=1  v_nominal_unit=V  vc_specify=off  vc_priority=High  vc=0 V  vc_nominal_specify=off  vc_nominal_value=1  vc_nominal_unit=V
  Inductor : fl_lib/Electrical/Electrical Elements/Inductor  l=1e-6 H  r=0 Ohm  g=1e-9 1/Ohm  i_specify=on  i_priority=High  i=0 A  i_nominal_specify=off  i_nominal_value=1  i_nominal_unit=A  v_specify=off  v_priority=None  v=0 V  v_nominal_specify=off  v_nominal_value=1  v_nominal_unit=V  i_L_specify=off  i_L_priority=High  i_L=0 A  i_L_nominal_specify=off  i_L_nominal_value=1  i_L_nominal_unit=A
  Inductor1 : fl_lib/Electrical/Electrical Elements/Inductor  l=1e-6 H  r=0 Ohm  g=1e-9 1/Ohm  i_specify=on  i_priority=High  i=0 A  i_nominal_specify=off  i_nominal_value=1  i_nominal_unit=A  v_specify=off  v_priority=None  v=0 V  v_nominal_specify=off  v_nominal_value=1  v_nominal_unit=V  i_L_specify=off  i_L_priority=High  i_L=0 A  i_L_nominal_specify=off  i_L_nominal_value=1  i_L_nominal_unit=A
  Inductor2 : fl_lib/Electrical/Electrical Elements/Inductor  l=1e-6 H  r=0 Ohm  g=1e-9 1/Ohm  i_specify=on  i_priority=High  i=0 A  i_nominal_specify=off  i_nominal_value=1  i_nominal_unit=A  v_specify=off  v_priority=None  v=0 V  v_nominal_specify=off  v_nominal_value=1  v_nominal_unit=V  i_L_specify=off  i_L_priority=High  i_L=0 A  i_L_nominal_specify=off  i_L_nominal_value=1  i_L_nominal_unit=A
  threephase inductor : threephase_inductor_lib/threephase inductor  Lp=hwdata.afe.LFu H  L0=hwdata.afe.LFu_cm H  Rp=hwdata.afe.RLFu Ohm  R0=hwdata.afe.RLFu_cm Ohm  Lls=5e-6 H  uu_1_specify=off  uu_1_priority=None  uu_1=0 V  uu_1_nominal_specify=off  uu_1_nominal_value=1  uu_1_nominal_unit=V  uv_1_specify=off  uv_1_priority=None  uv_1=0 V  uv_1_nominal_specify=off  uv_1_nominal_value=1  uv_1_nominal_unit=V  uw_1_specify=off  uw_1_priority=None  uw_1=0 V  uw_1_nominal_specify=off  uw_1_nominal_value=1  uw_1_nominal_unit=V  uu_2_specify=off  uu_2_priority=None  uu_2=0 V  uu_2_nominal_specify=off  uu_2_nominal_value=1  uu_2_nominal_unit=V  uv_2_specify=off  uv_2_priority=None  uv_2=0 V  uv_2_nominal_specify=off  uv_2_nominal_value=1  uv_2_nominal_unit=V  uw_2_specify=off  uw_2_priority=None  uw_2=0 V  uw_2_nominal_specify=off  uw_2_nominal_value=1  uw_2_nominal_unit=V  iu_specify=off  iu_priority=High  iu=0 A  iu_nominal_specify=off  iu_nominal_value=1  iu_nominal_unit=A  iv_specify=off  iv_priority=High  iv=0 A  iv_nominal_specify=off  iv_nominal_value=1  iv_nominal_unit=A  iw_specify=off  iw_priority=High  iw=0 A  iw_nominal_specify=off  iw_nominal_value=1  iw_nominal_unit=A
  threephase_vi_measures_grid : Subsystem
  threephase_vi_measures_stack : Subsystem
  us_a : PMIOPort  Side=Left
  ug_a : PMIOPort  Port=2  Side=Right
  us_b : PMIOPort  Port=3  Side=Left
  ug_b : PMIOPort  Port=4  Side=Right
  us_c : PMIOPort  Port=5  Side=Left
  ug_c : PMIOPort  Port=6  Side=Right
  connections:
  CFu1/RConn1 -- CFu3/RConn1 -- CFu2/RConn1
  Inductor/RConn1 -- threephase_vi_measures_grid/RConn1 -- CFu1/LConn1
  Inductor2/RConn1 -- threephase_vi_measures_grid/RConn3 -- CFu3/LConn1
  Inductor1/RConn1 -- threephase_vi_measures_grid/RConn2 -- CFu2/LConn1
  threephase_vi_measures_stack/RConn1 -- us_a/RConn1
  threephase_vi_measures_stack/RConn2 -- us_b/RConn1
  threephase_vi_measures_stack/RConn3 -- us_c/RConn1
  threephase_vi_measures_stack/LConn1 -- threephase inductor/LConn1
  threephase_vi_measures_stack/LConn2 -- threephase inductor/LConn2
  threephase_vi_measures_stack/LConn3 -- threephase inductor/LConn3
  threephase inductor/RConn1 -- Inductor/LConn1
  Inductor1/LConn1 -- threephase inductor/RConn2
  Inductor2/LConn1 -- threephase inductor/RConn3
  threephase_vi_measures_grid/LConn1 -- ug_a/RConn1
  threephase_vi_measures_grid/LConn2 -- ug_b/RConn1
  threephase_vi_measures_grid/LConn3 -- ug_c/RConn1

== system afe_inv_ttype_psm/afe_abc_inv_psm_mod1/afe ==
  dabc : Inport
  Bus Selector : BusSelector  OutputSignals=vdc_pu,udc,udc1,udc2,np_current,udc_p_gnd,udc_n_gnd,udc_centertap_gnd,Cdc1_current,Cdc2_current
  dclink : dclink_for_three_levels/dclink  Cdc1_m=hwdata.afe.CFi1  Cdc2_m=hwdata.afe.CFi2  Rudc_measure=107e3  Vdc_scale=hwdata.afe.udc_nom  Vdc1_m_init=hwdata.afe.udc_nom/2  Vdc2_m_init=hwdata.afe.udc_nom/2
  deadtime_generator_for_ttype : Subsystem
  ideal_switch_based_three_level_inverter_ttype : three_phase_three_level_ttype_inverter_ideal_switch_based_model/ideal_switch_based_three_level_inverter_ttype  Vth=5.5  Ron=1.5e-3  Vdon_diode=2  Rdon_diode=0.15e-3  Csnubber=10e-9  Rsnubber=2200
  sv_pwm : Subsystem
  udc_scope : Scope  NumInputPorts=2
      settings: ActiveDisplayYMinimum=-0.15179654734884226  ActiveDisplayYMaximum=1.3559215765150121  DataLoggingVariableName=ScopeData35
  us_a : PMIOPort  Side=Left
  us_b : PMIOPort  Port=2  Side=Left
  us_c : PMIOPort  Port=3  Side=Left
  Udc(+) : PMIOPort  Port=4  Side=Right
  Np : PMIOPort  Port=5  Side=Right
  Udc(-) : PMIOPort  Port=6  Side=Right
  tag scope: Cdc1_current=global, Cdc2_current=global, np_current=global, udc1=global, udc2=global, udc=global, udc_centertap_gnd=global, udc_n_gnd=global, udc_p_gnd=global, vdc_pu=global
  wires:
  Bus Selector/5 -> [np_current]  "<np_current>"
  [vdc_pu] -> udc_scope/2  "udc_pu"
  Bus Selector/8 -> [udc_centertap_gnd]  "<udc_centertap_gnd>"
  Bus Selector/10 -> [Cdc2_current]  "<Cdc2_current>"
  [udc] -> udc_scope/1  "udc"
  Bus Selector/1 -> [vdc_pu]  "<vdc_pu>"
  Bus Selector/7 -> [udc_n_gnd]  "<udc_n_gnd>"
  Bus Selector/9 -> [Cdc1_current]  "<Cdc1_current>"
  Bus Selector/3 -> [udc1]  "<udc1>"
  Bus Selector/4 -> [udc2]  "<udc2>"
  Bus Selector/6 -> [udc_p_gnd]  "<udc_p_gnd>"
  dclink/1 -> Bus Selector/1
  Bus Selector/2 -> [udc]  "<udc>"
  dabc/1 -> sv_pwm/1(duties_uvw)
  sv_pwm/1(gate_cmds) -> deadtime_generator_for_ttype/1(gate_cmds_in)
  deadtime_generator_for_ttype/1(gate_cmds_out) -> ideal_switch_based_three_level_inverter_ttype/1
  connections:
  dclink/RConn1 -- Udc(+)/RConn1
  dclink/RConn3 -- Udc(-)/RConn1
  ideal_switch_based_three_level_inverter_ttype/LConn3 -- us_c/RConn1
  dclink/RConn2 -- Np/RConn1
  dclink/LConn1 -- ideal_switch_based_three_level_inverter_ttype/RConn1
  ideal_switch_based_three_level_inverter_ttype/RConn3 -- dclink/LConn3
  ideal_switch_based_three_level_inverter_ttype/RConn2 -- dclink/LConn2
  us_b/RConn1 -- ideal_switch_based_three_level_inverter_ttype/LConn2
  ideal_switch_based_three_level_inverter_ttype/LConn1 -- us_a/RConn1

== system afe_inv_ttype_psm/afe_abc_inv_psm_mod1/brake ==
  Constant1 : Constant  Value=hwdata.afe.udc_nom
  Current Sensor3 : fl_lib/Electrical/Electrical Sensors/Current Sensor
  Integrator : Integrator
  MATLAB Function : MATLAB Function  TreatAsAtomicUnit=on  SystemSampleTime=glb_time.ts_afe
  PS-Simulink Converter : nesl_utility/PS-Simulink Converter  PhysicalDomain=network_engine_domain  SubClassName=ps_output  LeftPortType=input  RightPortType=output  PseudoPeriodic=off  Frequencies=[]  VectorFormat=1-D array  Unit=V  AffineConversion=off
  Product : Product
  Product6 : Product
  Rbrake : Subsystem
  Rbrake mod1 : Scope  NumInputPorts=2
      settings: SampleTime=glb_time.tc  ActiveDisplayYMinimum=-48635.262164896827  ActiveDisplayYMaximum=437717.35948407149  DataLoggingVariableName=ScopeData2
  Simulink-PS Converter4 : nesl_utility/Simulink-PS Converter  PhysicalDomain=network_engine_domain  SubClassName=ps_input  LeftPortType=input  RightPortType=output  PseudoPeriodic=off  Frequencies=[]  NoiseDistribution=none  NoiseParameters=[]  Unit=1  AffineConversion=on  FilteringAndDerivatives=provide  SimscapeFilterOrder=1  InputFilterTimeConstant=0.001  UdotUserProvided=0
  Step : Step  Time=time_aux_power_supply_fault  InitialValue=1  FinalValue=0  SampleTime=0
  To Workspace1 : ToWorkspace  VariableName=energy_Rbrake_sim_mod1  SampleTime=glb_time.tc
      settings: MaxDataPoints=glb_time.Nc
  To Workspace10 : ToWorkspace  VariableName=power_Rbrake_sim_mod1  SampleTime=glb_time.tc
      settings: MaxDataPoints=glb_time.Nc
  Unit Delay : UnitDelay  SampleTime=glb_time.ts_afe
  Voltage Sensor : fl_lib/Electrical/Electrical Sensors/Voltage Sensor
  Voltage Sensor1 : fl_lib/Electrical/Electrical Sensors/Voltage Sensor
  ibrakeR : nesl_utility/PS-Simulink Converter  PhysicalDomain=network_engine_domain  SubClassName=ps_output  LeftPortType=input  RightPortType=output  PseudoPeriodic=off  Frequencies=[]  VectorFormat=1-D array  Unit=A  AffineConversion=off
  switch_1 : Subsystem
      settings: PortSchema="{\"entries\":[{\"content\":{\"sides\":[{\"content\":{},\"type\":\"ConnectorPlacement.EquallySpacedRectSide\",\"uuid\":\"9277da8d-d460-43e6-8478-dd662f15d226\"},{\"content\":{\"side\":\"RIGHT\"},\"type\":\"ConnectorPlacement.EquallySpacedRectSide\",\"uuid\":\"a7ece396-f1d9-4f4f-a05b-db1fc65d6e1d\"},{\"content\":{\"connectorIds\":[\"LConn1\"],\"side\":\"TOP\"},\"type\":\"ConnectorPlacement.EquallySpacedRectSide\",\"uuid\":\"fdd70777-e9cf-4317-afb6-cae87f75d5b0\"},{\"content\":{\"connectorIds\":[\"RConn1\"],\"side\":\"BOTTOM\"},\"type\":\"ConnectorPlacement.EquallySpacedRectSide\",\"uuid\":\"2353ed68-b1a1-4775-9ca9-31e268d5443b\"}]},\"type\":\"ConnectorPlacement.EquallySpacedConnector\",\"uuid\":\"d5479f4c-4e65-4791-adcb-73df11f88590\"}],\"packageUris\":[\"http://schema.mathworks.com/mf0/Connector/R2020b\"],\"version\":\"1.0\"}"
  switch_2 : Subsystem
      settings: PortSchema="{\"entries\":[{\"content\":{\"sides\":[{\"content\":{\"connectorIds\":[\"LConn1\"]},\"type\":\"ConnectorPlacement.EquallySpacedRectSide\",\"uuid\":\"9277da8d-d460-43e6-8478-dd662f15d226\"},{\"content\":{\"connectorIds\":[],\"side\":\"RIGHT\"},\"type\":\"ConnectorPlacement.EquallySpacedRectSide\",\"uuid\":\"a7ece396-f1d9-4f4f-a05b-db1fc65d6e1d\"},{\"content\":{\"connectorIds\":[\"LConn2\"],\"side\":\"TOP\"},\"type\":\"ConnectorPlacement.EquallySpacedRectSide\",\"uuid\":\"fdd70777-e9cf-4317-afb6-cae87f75d5b0\"},{\"content\":{\"connectorIds\":[\"RConn1\"],\"side\":\"BOTTOM\"},\"type\":\"ConnectorPlacement.EquallySpacedRectSide\",\"uuid\":\"2353ed68-b1a1-4775-9ca9-31e268d5443b\"}]},\"type\":\"ConnectorPlacement.EquallySpacedConnector\",\"uuid\":\"d5479f4c-4e65-4791-adcb-73df11f88590\"}],\"packageUris\":[\"http://schema.mathworks.com/mf0/Connector/R2020b\"],\"version\":\"1.0\"}"
  ubrakeR : nesl_utility/PS-Simulink Converter  PhysicalDomain=network_engine_domain  SubClassName=ps_output  LeftPortType=input  RightPortType=output  PseudoPeriodic=off  Frequencies=[]  VectorFormat=1-D array  Unit=V  AffineConversion=off
  dc(+) : PMIOPort  Side=Left
  dc(-) : PMIOPort  Port=2  Side=Left
  tag scope: energy_Rbrake_mod1=global, power_Rbrake_mod1=global
  wires:
  Constant1/1 -> MATLAB Function/2(udc_ref)
  PS-Simulink Converter/1 -> MATLAB Function/1(u)
  MATLAB Function/1(y) -> Unit Delay/1
  ibrakeR/1 -> Product/1  "ibrakeR"
  ubrakeR/1 -> Product/2  "ubrakeR"
  Product/1 -> [power_Rbrake_mod1], Integrator/1
  Integrator/1 -> [energy_Rbrake_mod1]
  [power_Rbrake_mod1] -> To Workspace10/1, Rbrake mod1/1  "power_Rbrake"
  [energy_Rbrake_mod1] -> To Workspace1/1, Rbrake mod1/2  "energy_Rbrake"
  Step/1 -> Product6/1
  Unit Delay/1 -> Product6/2
  Product6/1 -> Simulink-PS Converter4/1
  connections:
  dc(-)/RConn1 -- switch_2/RConn1 -- Voltage Sensor/RConn2
  switch_1/RConn1 -- Voltage Sensor1/RConn2 -- Rbrake/RConn1 -- switch_2/LConn2
  PS-Simulink Converter/LConn1 -- Voltage Sensor/RConn1
  switch_2/LConn1 -- Simulink-PS Converter4/RConn1
  Voltage Sensor/LConn1 -- Current Sensor3/LConn1 -- switch_1/LConn1 -- dc(+)/RConn1
  Current Sensor3/RConn1 -- ibrakeR/LConn1
  Voltage Sensor1/RConn1 -- ubrakeR/LConn1
  Current Sensor3/RConn2 -- Voltage Sensor1/LConn1 -- Rbrake/LConn1

== system afe_inv_ttype_psm/afe_abc_inv_psm_mod1/inv_psm_mod1 ==
  Goto Tag Visibility : GotoTagVisibility  GotoTag=vdc_pu
  Goto Tag Visibility1 : GotoTagVisibility  GotoTag=udc
  Goto Tag Visibility10 : GotoTagVisibility  GotoTag=udc1_pu
  Goto Tag Visibility11 : GotoTagVisibility  GotoTag=udc2_pu
  Goto Tag Visibility2 : GotoTagVisibility  GotoTag=udc1
  Goto Tag Visibility3 : GotoTagVisibility  GotoTag=udc2
  Goto Tag Visibility4 : GotoTagVisibility  GotoTag=np_current
  Goto Tag Visibility5 : GotoTagVisibility  GotoTag=udc_p_gnd
  Goto Tag Visibility6 : GotoTagVisibility  GotoTag=udc_n_gnd
  Goto Tag Visibility7 : GotoTagVisibility  GotoTag=udc_centertap_gnd
  Goto Tag Visibility8 : GotoTagVisibility  GotoTag=Cdc1_current
  Goto Tag Visibility9 : GotoTagVisibility  GotoTag=Cdc2_current
  dclink : Subsystem
  inverter : Subsystem
  inverter_ctrl : Subsystem
  inverter_output_filter : Subsystem
  us_u : PMIOPort  Side=Right
  us_v : PMIOPort  Port=2  Side=Right
  us_w : PMIOPort  Port=3  Side=Right
  udc(+) : PMIOPort  Port=4  Side=Left
  np : PMIOPort  Port=5  Side=Left
  udc(-) : PMIOPort  Port=6  Side=Left
  wires:
  inverter_ctrl/1(cmd_gates) -> inverter/1(gate_cmds_uvw)
  connections:
  inverter_output_filter/LConn2 -- us_v/RConn1
  inverter_output_filter/LConn3 -- us_w/RConn1
  inverter_output_filter/LConn1 -- us_u/RConn1
  dclink/LConn1 -- udc(+)/RConn1
  dclink/LConn3 -- udc(-)/RConn1
  inverter/RConn2 -- dclink/RConn2
  inverter/RConn1 -- dclink/RConn1
  inverter/RConn3 -- dclink/RConn3
  inverter_output_filter/RConn3 -- inverter/LConn3
  inverter_output_filter/RConn2 -- inverter/LConn2
  inverter_output_filter/RConn1 -- inverter/LConn1
  np/RConn1 -- dclink/LConn2

== system afe_inv_ttype_psm/global timing/time_afe1 ==
  correction_time : Inport
  Constant : Constant
  Gain : Gain  Gain=k
  Product : Product
  Sum : Sum  Inputs=|++
  time_1 : Clock
  Out1 : Outport
  wires:
  time_1/1 -> Gain/1
  Gain/1 -> Product/1
  Product/1 -> Out1/1
  correction_time/1 -> Sum/1
  Sum/1 -> Product/2
  Constant/1 -> Sum/2
